simulink model "nmm2d"  (R2025a)
settings: Solver=ode15s  StartTime=0.0  StopTime=20  FixedStep=1e-3  MaxStep=ts_max  RelTol=1e-3  AbsTol=1e-4  EnableMultiTasking=on
values from neighbouring files (symbols this model uses):
  c = 0.05    [nmm2d_mInit.m]
  c_jointstop = 0.3 / (pi/180)    (= 17.1887338539)    [nmm2d_mInit.m]
  D12_F = 0.16    [nmm2d_mInit.m]
  D12_S = L_S    (= 0.5)    [nmm2d_mInit.m]
  D12_T = L_T    (= 0.5)    [nmm2d_mInit.m]
  D1G_F = 0.14    [nmm2d_mInit.m]
  D1G_HAT = 0.35    [nmm2d_mInit.m]
  D1G_S = 0.3    [nmm2d_mInit.m]
  D1G_T = 0.3    [nmm2d_mInit.m]
  DeltaThRef = 5e-3    (= 0.005)    [nmm2d_mInit.m]
  eref = 0.04    [nmm2d_mInit.m]
  FmaxVec = [FmaxSOL FmaxTA FmaxGAS FmaxVAS FmaxHAM FmaxGLU FmaxHFL               FmaxSOL FmaxTA FmaxGAS FmaxVAS FmaxHAM FmaxGLU FmaxHFL]'    [nmm2d_mInit.m]
  g = 9.81    [nmm2d_mInit.m]
  GainDeltaTheta = 2 /100*180/pi    (= 1.14591559026)    [nmm2d_cInit.m]
  GainGAS = 1.1/FmaxGAS    [nmm2d_cInit.m]
  GainGLU = 0.5/FmaxGLU    [nmm2d_cInit.m]
  GainHAM = 0.65/FmaxHAM    [nmm2d_cInit.m]
  GainHAMHFL = 4    [nmm2d_cInit.m]
  GainHFL = 0.5    [nmm2d_cInit.m]
  GainKneOverExt = 2    [nmm2d_cInit.m]
  GainSOL = 1.2/FmaxSOL    [nmm2d_cInit.m]
  GainSOLTA = 0.4/FmaxSOL    [nmm2d_cInit.m]
  GainTA = 1.1    [nmm2d_cInit.m]
  GainVAS = 1.2/FmaxVAS    [nmm2d_cInit.m]
  HAT_CG0 = [-D12_F; 0] + Rot120*[L_S;0] + Rot120*Rot230*[-L_T;0]            + Rot120*Rot230*Rot340*[D1G_HAT;0]    [nmm2d_cInit.m]
  In_F = 0.005    [nmm2d_mInit.m]
  In_HAT = 3    [nmm2d_mInit.m]
  In_S = 0.05    [nmm2d_mInit.m]
  In_T = 0.15    [nmm2d_mInit.m]
  K = 5    [nmm2d_mInit.m]
  k_gx = (2*(m_F+m_S+m_T)+m_HAT)*g/0.1    (= 7848)    [nmm2d_mInit.m]
  k_gy = (2*(m_F+m_S+m_T)+m_HAT)*g/0.01    (= 78480)    [nmm2d_mInit.m]
  k_pressure = m_HAT * 9.81 / DeltaThRef    (= 104967)    [nmm2d_mInit.m]
  K_swing = 0.25    [nmm2d_cInit.m]
  KneePh23Offset = 170*pi/180    (= 2.96705972839)    [nmm2d_cInit.m]
  L_F = 0.2    [nmm2d_mInit.m]
  L_HAT = 0.8    [nmm2d_mInit.m]
  L_S = 0.5    [nmm2d_mInit.m]
  L_T = 0.5    [nmm2d_mInit.m]
  LceOffsetHAM = 0.85    [nmm2d_cInit.m]
  LceOffsetHFL = 0.65    [nmm2d_cInit.m]
  LceOffsetTA = 1-0.5*w    [nmm2d_cInit.m]
  LongDelay = 0.020    (= 0.02)    [nmm2d_cInit.m]
  loptGAS = 0.05    [nmm2d_mInit.m]
  loptGLU = 0.11    [nmm2d_mInit.m]
  loptHAM = 0.10    (= 0.1)    [nmm2d_mInit.m]
  loptHFL = 0.11    [nmm2d_mInit.m]
  loptSOL = 0.04    [nmm2d_mInit.m]
  loptTA = 0.06    [nmm2d_mInit.m]
  loptVAS = 0.08    [nmm2d_mInit.m]
  loptVec = [loptSOL loptTA loptGAS loptVAS loptHAM loptGLU loptHFL               loptSOL loptTA loptGAS loptVAS loptHAM loptGLU loptHFL]'    [nmm2d_mInit.m]
  Lphi120 = 85*pi/180    (= 1.4835298642)    [nmm2d_cInit.m]
  Lphi230 = 175*pi/180    (= 3.05432619099)    [nmm2d_cInit.m]
  Lphi340 = 175*pi/180    (= 3.05432619099)    [nmm2d_cInit.m]
  lslackGAS = 0.40    (= 0.4)    [nmm2d_mInit.m]
  lslackGLU = 0.13    [nmm2d_mInit.m]
  lslackHAM = 0.31    [nmm2d_mInit.m]
  lslackHFL = 0.10    (= 0.1)    [nmm2d_mInit.m]
  lslackSOL = 0.26    [nmm2d_mInit.m]
  lslackTA = 0.24    [nmm2d_mInit.m]
  lslackVAS = 0.23    [nmm2d_mInit.m]
  lslackVec = [lslackSOL lslackTA lslackGAS lslackVAS lslackHAM lslackGLU lslackHFL                 lslackSOL lslackTA lslackGAS lslackVAS lslackHAM lslackGLU lslackHFL]'    [nmm2d_mInit.m]
  m_F = 1.25    [nmm2d_mInit.m]
  m_HAT = 53.5    [nmm2d_mInit.m]
  m_S = 3.5    [nmm2d_mInit.m]
  m_T = 8.5    [nmm2d_mInit.m]
  MidDelay = 0.010    (= 0.01)    [nmm2d_cInit.m]
  mu_slide = 0.8    [nmm2d_mInit.m]
  mu_stick = 0.9    [nmm2d_mInit.m]
  N = 1.5    [nmm2d_mInit.m]
  phi12_LowLimit = 70*pi/180    (= 1.2217304764)    [nmm2d_mInit.m]
  phi12_UpLimit = 130*pi/180    (= 2.26892802759)    [nmm2d_mInit.m]
  phi23_UpLimit = 175*pi/180    (= 3.05432619099)    [nmm2d_mInit.m]
  phi34_UpLimit = 230*pi/180    (= 4.01425727959)    [nmm2d_mInit.m]
  phimaxGASa = 110*pi/180    (= 1.91986217719)    [nmm2d_mInit.m]
  phimaxGASk = 140*pi/180    (= 2.44346095279)    [nmm2d_mInit.m]
  phimaxHAMk = 180*pi/180    (= 3.14159265359)    [nmm2d_mInit.m]
  phimaxSOL = 110*pi/180    (= 1.91986217719)    [nmm2d_mInit.m]
  phimaxTA = 80*pi/180    (= 1.3962634016)    [nmm2d_mInit.m]
  phimaxVAS = 165*pi/180    (= 2.87979326579)    [nmm2d_mInit.m]
  phirefGASa = 80*pi/180    (= 1.3962634016)    [nmm2d_mInit.m]
  phirefGASk = 165*pi/180    (= 2.87979326579)    [nmm2d_mInit.m]
  phirefGLU = 150*pi/180    (= 2.61799387799)    [nmm2d_mInit.m]
  phirefHAMh = 155*pi/180    (= 2.70526034059)    [nmm2d_mInit.m]
  phirefHAMk = 180*pi/180    (= 3.14159265359)    [nmm2d_mInit.m]
  phirefHFL = 180*pi/180    (= 3.14159265359)    [nmm2d_mInit.m]
  phirefSOL = 80*pi/180    (= 1.3962634016)    [nmm2d_mInit.m]
  phirefTA = 110*pi/180    (= 1.91986217719)    [nmm2d_mInit.m]
  phirefVAS = 125*pi/180    (= 2.18166156499)    [nmm2d_mInit.m]
  PosGainGG = 1/(30*pi/180)    (= 1.9098593171)    [nmm2d_cInit.m]
  preA = 0.01    [nmm2d_mInit.m]
  PreStimGAS = 0.01    [nmm2d_cInit.m]
  PreStimGG = 0.05    [nmm2d_cInit.m]
  PreStimGLU = 0.01    [nmm2d_cInit.m]
  PreStimHAM = 0.01    [nmm2d_cInit.m]
  PreStimHFL = 0.01    [nmm2d_cInit.m]
  PreStimSOL = 0.01    [nmm2d_cInit.m]
  PreStimTA = 0.01    [nmm2d_cInit.m]
  PreStimVAS = 0.08    [nmm2d_cInit.m]
  rGASa = 0.05    [nmm2d_mInit.m]
  rGASk = 0.05    [nmm2d_mInit.m]
  rGLU = 0.10    (= 0.1)    [nmm2d_mInit.m]
  rHAMh = 0.08    [nmm2d_mInit.m]
  rHAMk = 0.05    [nmm2d_mInit.m]
  rHFL = 0.10    (= 0.1)    [nmm2d_mInit.m]
  rhoGASa = 0.7    [nmm2d_mInit.m]
  rhoGASk = 0.7    [nmm2d_mInit.m]
  rhoGLU = 0.5    [nmm2d_mInit.m]
  rhoHAMh = 0.7    [nmm2d_mInit.m]
  rhoHAMk = 0.7    [nmm2d_mInit.m]
  rhoHFL = 0.5    [nmm2d_mInit.m]
  rhoSOL = 0.5    [nmm2d_mInit.m]
  rhoTA = 0.7    [nmm2d_mInit.m]
  rhoVAS = 0.7    [nmm2d_mInit.m]
  Rphi120 = 90*pi/180    (= 1.57079632679)    [nmm2d_cInit.m]
  Rphi230 = 175*pi/180    (= 3.05432619099)    [nmm2d_cInit.m]
  Rphi340 = 140*pi/180    (= 2.44346095279)    [nmm2d_cInit.m]
  rSOL = 0.05    [nmm2d_mInit.m]
  rTA = 0.04    [nmm2d_mInit.m]
  rVAS = 0.06    [nmm2d_mInit.m]
  ... (+12 more)
undefined symbols (not defined in the file or in its folder): sgn, X, Y, Z
libraries: sm_lib x70, nesl_utility x67, simulink x27, simulink_extras x6
(part 4 of 5)

== system nmm2d/Body Mechanics Layer/body sensor2 ==
  Frame Sensor : sm_lib/Frames and Transforms/Transform Sensor  MeasurementFrame=World  RotationSequence=XYX  SenseAngle=off  SenseAxis=off  SenseQ=off  SenseR=off  SenseRotationSequence=off  SenseOmegaX=off  SenseOmegaY=off  SenseOmegaZ=off  SenseOmega=off  SenseQDot=off  SenseRDot=off  SenseRotationSequenceDot=off  SenseAlphaX=off  SenseAlphaY=off  SenseAlphaZ=off  SenseAlpha=off  SenseQDDot=off  SenseRDDot=off  SenseX=on  SenseY=on  SenseZ=on  SenseXYZ=off  SenseRad=off  SenseAzim=off  SenseDist=off  SenseInc=off  SenseXDot=on  SenseYDot=on  SenseZDot=on  SenseXYZDot=off  SenseRadDot=off  SenseAzimDot=off  SenseDistDot=off  SenseIncDot=off  SenseXDDot=off  SenseYDDot=off  SenseZDDot=off  SenseXYZDDot=off  SenseRadDDot=off  SenseAzimDDot=off  SenseDistDDot=off  SenseIncDDot=off
  Mux : Mux  Inputs=3
  Mux1 : Mux  Inputs=3
  PS-Simulink Converter : nesl_utility/PS-Simulink Converter  PhysicalDomain=network_engine_domain  SubClassName=ps_output  LeftPortType=input  RightPortType=output  PseudoPeriodic=off  Frequencies=[]  VectorFormat=1-D array  Unit=m  AffineConversion=off
  PS-Simulink Converter1 : nesl_utility/PS-Simulink Converter  PhysicalDomain=network_engine_domain  SubClassName=ps_output  LeftPortType=input  RightPortType=output  PseudoPeriodic=off  Frequencies=[]  VectorFormat=1-D array  Unit=m  AffineConversion=off
  PS-Simulink Converter2 : nesl_utility/PS-Simulink Converter  PhysicalDomain=network_engine_domain  SubClassName=ps_output  LeftPortType=input  RightPortType=output  PseudoPeriodic=off  Frequencies=[]  VectorFormat=1-D array  Unit=m/s  AffineConversion=off
  PS-Simulink Converter3 : nesl_utility/PS-Simulink Converter  PhysicalDomain=network_engine_domain  SubClassName=ps_output  LeftPortType=input  RightPortType=output  PseudoPeriodic=off  Frequencies=[]  VectorFormat=1-D array  Unit=m/s  AffineConversion=off
  PS-Simulink Converter4 : nesl_utility/PS-Simulink Converter  PhysicalDomain=network_engine_domain  SubClassName=ps_output  LeftPortType=input  RightPortType=output  PseudoPeriodic=off  Frequencies=[]  VectorFormat=1-D array  Unit=m  AffineConversion=off
  PS-Simulink Converter5 : nesl_utility/PS-Simulink Converter  PhysicalDomain=network_engine_domain  SubClassName=ps_output  LeftPortType=input  RightPortType=output  PseudoPeriodic=off  Frequencies=[]  VectorFormat=1-D array  Unit=m/s  AffineConversion=off
  World Frame : sm_lib/Frames and Transforms/World Frame
  frame : PMIOPort  Side=Left
  p [m x3] : Outport
  v [m/s x3] : Outport  Port=2
  wires:
  PS-Simulink Converter1/1 -> Mux/2
  PS-Simulink Converter/1 -> Mux/1
  PS-Simulink Converter2/1 -> Mux1/1
  PS-Simulink Converter3/1 -> Mux1/2
  Mux1/1 -> v [m/s x3]/1
  Mux/1 -> p [m x3]/1
  PS-Simulink Converter4/1 -> Mux/3
  PS-Simulink Converter5/1 -> Mux1/3
  connections:
  Frame Sensor/RConn1 -- frame/RConn1
  World Frame/RConn1 -- Frame Sensor/LConn1
  Frame Sensor/RConn2 -- PS-Simulink Converter/LConn1
  PS-Simulink Converter1/LConn1 -- Frame Sensor/RConn3
  PS-Simulink Converter2/LConn1 -- Frame Sensor/RConn5
  PS-Simulink Converter3/LConn1 -- Frame Sensor/RConn6
  PS-Simulink Converter4/LConn1 -- Frame Sensor/RConn4
  PS-Simulink Converter5/LConn1 -- Frame Sensor/RConn7

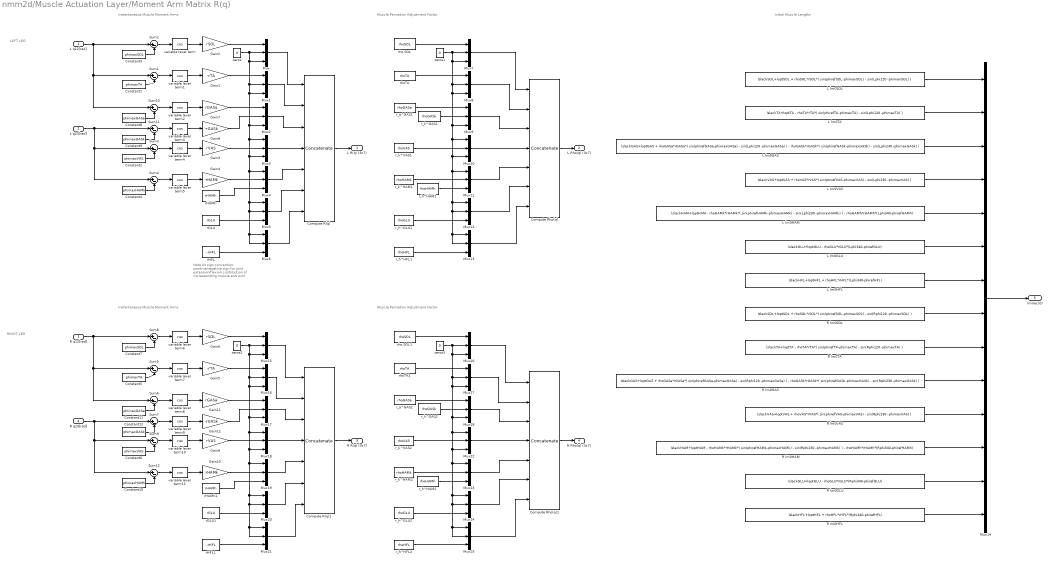
== system nmm2d/Muscle Actuation Layer/Moment Arm Matrix R(q) ==
  note: LEFT LEG
  note: Muscle Pennation Adjustment Factor
  note: Initial Muscle Lengths
  note: Instantaneous Muscle Moment Arms
  note: Note on sign convention:
      | positive/negative sign for
      | joint extension/flexion contribution
      | of corresponding muscle and joint
  note: Instantaneous Muscle Moment Arms
  note: RIGHT LEG
  note: Muscle Pennation Adjustment Factor
  L q12[rad] : Inport
  L q23[rad] : Inport  Port=2
  R q12[rad] : Inport  Port=3
  R q23[rad] : Inport  Port=4
  Compute R(q) : Concatenate  NumInputs=7  Mode=Multidimensional array  ConcatenateDimension=2
  Compute R(q)1 : Concatenate  NumInputs=7  Mode=Multidimensional array  ConcatenateDimension=2
  Compute Rho(q) : Concatenate  NumInputs=7  Mode=Multidimensional array  ConcatenateDimension=2
  Compute Rho(q)1 : Concatenate  NumInputs=7  Mode=Multidimensional array  ConcatenateDimension=2
  Constant1 : Constant  Value=phimaxTA
  Constant10 : Constant  Value=phimaxHAMk
  Constant11 : Constant  Value=phimaxGASa
  Constant12 : Constant  Value=phimaxGASk
  Constant2 : Constant  Value=phimaxVAS
  Constant3 : Constant  Value=phimaxSOL
  Constant4 : Constant  Value=phimaxHAMk
  Constant5 : Constant  Value=phimaxTA
  Constant6 : Constant  Value=phimaxVAS
  Constant7 : Constant  Value=phimaxSOL
  Constant8 : Constant  Value=phimaxGASa
  Constant9 : Constant  Value=phimaxGASk
  Gain1 : Gain  Gain=-rTA
  Gain10 : Gain  Gain=-rHAMk
  Gain11 : Gain  Gain=rGASa
  Gain12 : Gain  Gain=-rGASk
  Gain2 : Gain  Gain=rSOL
  Gain3 : Gain  Gain=rVAS
  Gain4 : Gain  Gain=-rHAMk
  Gain5 : Gain  Gain=-rTA
  Gain6 : Gain  Gain=rSOL
  Gain7 : Gain  Gain=rGASa
  Gain8 : Gain  Gain=-rGASk
  Gain9 : Gain  Gain=rVAS
  L lm0GAS : Constant  Value=lslackGAS+loptGAS + rhoGASa*rGASa*( sin(phirefGASa-phimaxGASa) - sin(Lphi120 -phimaxGASa) ) - rhoGASk*rGASk*( sin(phirefGASk-phimaxGASk) - sin(Lphi230 -phimaxGASk) )
  L lm0GLU : Constant  Value=lslackGLU+loptGLU - rhoGLU*rGLU*(Lphi340-phirefGLU)
  L lm0HAM : Constant  Value=lslackHAM+loptHAM - rhoHAMk*rHAMk*( sin(phirefHAMk-phimaxHAMk) - sin(Lphi230 -phimaxHAMk) ) - rhoHAMh*rHAMh*(Lphi340-phirefHAMh)
  L lm0HFL : Constant  Value=lslackHFL+loptHFL + rhoHFL*rHFL*(Lphi340-phirefHFL)
  L lm0SOL : Constant  Value=lslackSOL+loptSOL + rhoSOL*rSOL*( sin(phirefSOL-phimaxSOL) - sin(Lphi120 -phimaxSOL) )
  L lm0TA : Constant  Value=lslackTA+loptTA - rhoTA*rTA*( sin(phirefTA-phimaxTA) - sin(Lphi120 -phimaxTA) )
  L lm0VAS : Constant  Value=lslackVAS+loptVAS + rhoVAS*rVAS*( sin(phirefVAS-phimaxVAS) - sin(Lphi230 -phimaxVAS) )
  Mux{,1..13,15..28} (28 alike) : Mux  Inputs=3
  Mux14 : Mux  Inputs=14
  R lm0GAS : Constant  Value=lslackGAS+loptGAS + rhoGASa*rGASa*( sin(phirefGASa-phimaxGASa) - sin(Rphi120 -phimaxGASa) ) - rhoGASk*rGASk*( sin(phirefGASk-phimaxGASk) - sin(Rphi230 -phimaxGASk) )
  R lm0GLU : Constant  Value=lslackGLU+loptGLU - rhoGLU*rGLU*(Rphi340-phirefGLU)
  R lm0HAM : Constant  Value=lslackHAM+loptHAM - rhoHAMk*rHAMk*( sin(phirefHAMk-phimaxHAMk) - sin(Rphi230 -phimaxHAMk) ) - rhoHAMh*rHAMh*(Rphi340-phirefHAMh)
  R lm0HFL : Constant  Value=lslackHFL+loptHFL + rhoHFL*rHFL*(Rphi340-phirefHFL)
  R lm0SOL : Constant  Value=lslackSOL+loptSOL + rhoSOL*rSOL*( sin(phirefSOL-phimaxSOL) - sin(Rphi120 -phimaxSOL) )
  R lm0TA : Constant  Value=lslackTA+loptTA - rhoTA*rTA*( sin(phirefTA-phimaxTA) - sin(Rphi120 -phimaxTA) )
  R lm0VAS : Constant  Value=lslackVAS+loptVAS + rhoVAS*rVAS*( sin(phirefVAS-phimaxVAS) - sin(Rphi230 -phimaxVAS) )
  Sum{1..12} (12 alike) : Sum  Inputs=|+-
  rGLU : Constant  Value=rGLU
  rGLU1 : Constant  Value=rGLU
  rHAMh : Constant  Value=rHAMh
  rHAMh1 : Constant  Value=rHAMh
  rHFL : Constant  Value=-rHFL
  rHFL1 : Constant  Value=-rHFL
  r_a^GAS1 : Constant  Value=rhoGASa
  r_a^GAS2 : Constant  Value=rhoGASa
  r_h^GLU1 : Constant  Value=rhoGLU
  r_h^GLU2 : Constant  Value=rhoGLU
  r_h^HAM1 : Constant  Value=rhoHAMh
  r_h^HAM2 : Constant  Value=rhoHAMh
  r_h^HFL1 : Constant  Value=rhoHFL
  r_h^HFL2 : Constant  Value=rhoHFL
  r_k^GAS1 : Constant  Value=rhoGASk
  r_k^GAS2 : Constant  Value=rhoGASk
  r_k^HAM1 : Constant  Value=rhoHAMk
  r_k^HAM2 : Constant  Value=rhoHAMk
  r_k^VAS1 : Constant  Value=rhoVAS
  r_k^VAS2 : Constant  Value=rhoVAS
  rho SOL : Constant  Value=rhoSOL
  rho SOL1 : Constant  Value=rhoSOL
  rhoTA : Constant  Value=rhoTA
  rhoTA1 : Constant  Value=rhoTA
  variable lever term{,1..11} (12 alike) : Trigonometry  Operator=cos
  zeros{,1..3} (4 alike) : Constant  Value=0
  L R(q) (3x7) : Outport
  L Rho(q) (3x7) : Outport  Port=2
  R R(q) (3x7) : Outport  Port=3
  R Rho(q) (3x7) : Outport  Port=4
  lmVec(0) : Outport  Port=5
  wires:
  Compute Rho(q)/1 -> L Rho(q) (3x7)/1
  rho SOL/1 -> Mux7/1
  Mux7/1 -> Compute Rho(q)/1
  r_k^GAS1/1 -> Mux9/2
  r_k^HAM1/1 -> Mux11/2
  r_k^VAS1/1 -> Mux10/2
  Mux13/1 -> Compute Rho(q)/7
  Mux8/1 -> Compute Rho(q)/2
  r_h^HAM1/1 -> Mux11/3
  Mux12/1 -> Compute Rho(q)/6
  r_h^GLU1/1 -> Mux12/3
  r_h^HFL1/1 -> Mux13/3
  Mux10/1 -> Compute Rho(q)/4
  rhoTA/1 -> Mux8/1
  Mux9/1 -> Compute Rho(q)/3
  zeros1/1 -> Mux7/2, Mux7/3, Mux8/2, Mux8/3, Mux9/3, Mux10/1, Mux10/3, Mux11/1, Mux12/1, Mux12/2, Mux13/2, Mux13/1
  r_a^GAS1/1 -> Mux9/1
  Mux11/1 -> Compute Rho(q)/5
  L lm0VAS/1 -> Mux14/4
  L lm0SOL/1 -> Mux14/1
  L lm0GAS/1 -> Mux14/3
  L q23[rad]/1 -> Sum11/1, Sum3/1, Sum4/1
  Sum4/1 -> variable lever term5/1
  Constant4/1 -> Sum4/2
  variable lever term5/1 -> Gain4/1
  Constant3/1 -> Sum2/2
  variable lever term/1 -> Gain2/1
  Constant2/1 -> Sum3/2
  variable lever term4/1 -> Gain3/1
  Mux/1 -> Compute R(q)/1
  Gain4/1 -> Mux4/2
  Mux6/1 -> Compute R(q)/7
  L lm0HAM/1 -> Mux14/5
  Gain2/1 -> Mux/1
  Sum3/1 -> variable lever term4/1
  Compute R(q)/1 -> L R(q) (3x7)/1
  Mux2/1 -> Compute R(q)/3
  Gain7/1 -> Mux2/1
  Mux5/1 -> Compute R(q)/6
  Gain8/1 -> Mux2/2
  Mux1/1 -> Compute R(q)/2
  rGLU/1 -> Mux5/3
  zeros/1 -> Mux/2, Mux/3, Mux1/2, Mux1/3, Mux2/3, Mux3/1, Mux3/3, Mux4/1, Mux5/1, Mux5/2, Mux6/2, Mux6/1
  Gain3/1 -> Mux3/2
  Mux4/1 -> Compute R(q)/5
  Sum2/1 -> variable lever term/1
  rHAMh/1 -> Mux4/3
  rHFL/1 -> Mux6/3
  Mux3/1 -> Compute R(q)/4
  Sum1/1 -> variable lever term1/1
  variable lever term1/1 -> Gain1/1
  Gain1/1 -> Mux1/1
  L lm0GLU/1 -> Mux14/6
  L lm0HFL/1 -> Mux14/7
  Mux14/1 -> lmVec(0)/1
  variable lever term3/1 -> Gain8/1
  L lm0TA/1 -> Mux14/2
  Constant9/1 -> Sum11/2
  L q12[rad]/1 -> Sum2/1, Sum1/1, Sum10/1
  variable lever term2/1 -> Gain7/1
  Constant8/1 -> Sum10/2
  Constant1/1 -> Sum1/2
  Sum10/1 -> variable lever term2/1
  Sum11/1 -> variable lever term3/1
  Gain10/1 -> Mux19/2
  Constant7/1 -> Sum8/2
  Sum6/1 -> variable lever term8/1
  rHAMh1/1 -> Mux19/3
  Sum9/1 -> variable lever term10/1
  Sum8/1 -> variable lever term6/1
  rHFL1/1 -> Mux21/3
  Constant5/1 -> Sum5/2
  variable lever term8/1 -> Gain11/1
  Gain5/1 -> Mux16/1
  zeros2/1 -> Mux21/1, Mux21/2, Mux20/2, Mux20/1, Mux19/1, Mux18/3, Mux18/1, Mux17/3, Mux16/3, Mux16/2, Mux15/3, Mux15/2
  variable lever term7/1 -> Gain5/1
  Gain12/1 -> Mux17/2
  variable lever term11/1 -> Gain10/1
  Constant11/1 -> Sum6/2
  Sum12/1 -> variable lever term11/1
  Constant6/1 -> Sum9/2
  variable lever term10/1 -> Gain9/1
  Gain11/1 -> Mux17/1
  variable lever term6/1 -> Gain6/1
  R q12[rad]/1 -> Sum6/1, Sum5/1, Sum8/1
  R q23[rad]/1 -> Sum12/1, Sum9/1, Sum7/1
  variable lever term9/1 -> Gain12/1
  Gain9/1 -> Mux18/2
  Sum7/1 -> variable lever term9/1
  Constant10/1 -> Sum12/2
  Gain6/1 -> Mux15/1
  Sum5/1 -> variable lever term7/1
  Constant12/1 -> Sum7/2
  rGLU1/1 -> Mux20/3
  r_a^GAS2/1 -> Mux28/1
  zeros3/1 -> Mux25/1, Mux25/2, Mux24/2, Mux24/1, Mux23/1, Mux22/3, Mux22/1, Mux28/3, Mux27/3, Mux27/2, Mux26/3, Mux26/2
  rhoTA1/1 -> Mux27/1
  r_h^HFL2/1 -> Mux25/3
  r_h^GLU2/1 -> Mux24/3
  r_h^HAM2/1 -> Mux23/3
  r_k^VAS2/1 -> Mux22/2
  r_k^HAM2/1 -> Mux23/2
  r_k^GAS2/1 -> Mux28/2
  rho SOL1/1 -> Mux26/1
  R lm0SOL/1 -> Mux14/8
  R lm0TA/1 -> Mux14/9
  R lm0VAS/1 -> Mux14/11
  R lm0GAS/1 -> Mux14/10
  R lm0HAM/1 -> Mux14/12
  R lm0GLU/1 -> Mux14/13
  R lm0HFL/1 -> Mux14/14
  Compute Rho(q)1/1 -> R Rho(q) (3x7)/1
  Mux22/1 -> Compute Rho(q)1/4
  Mux26/1 -> Compute Rho(q)1/1
  Mux27/1 -> Compute Rho(q)1/2
  Mux28/1 -> Compute Rho(q)1/3
  Mux23/1 -> Compute Rho(q)1/5
  Mux24/1 -> Compute Rho(q)1/6
  Mux25/1 -> Compute Rho(q)1/7
  Compute R(q)1/1 -> R R(q) (3x7)/1
  Mux18/1 -> Compute R(q)1/4
  Mux15/1 -> Compute R(q)1/1
  Mux16/1 -> Compute R(q)1/2
  Mux17/1 -> Compute R(q)1/3
  Mux19/1 -> Compute R(q)1/5
  Mux20/1 -> Compute R(q)1/6
  Mux21/1 -> Compute R(q)1/7

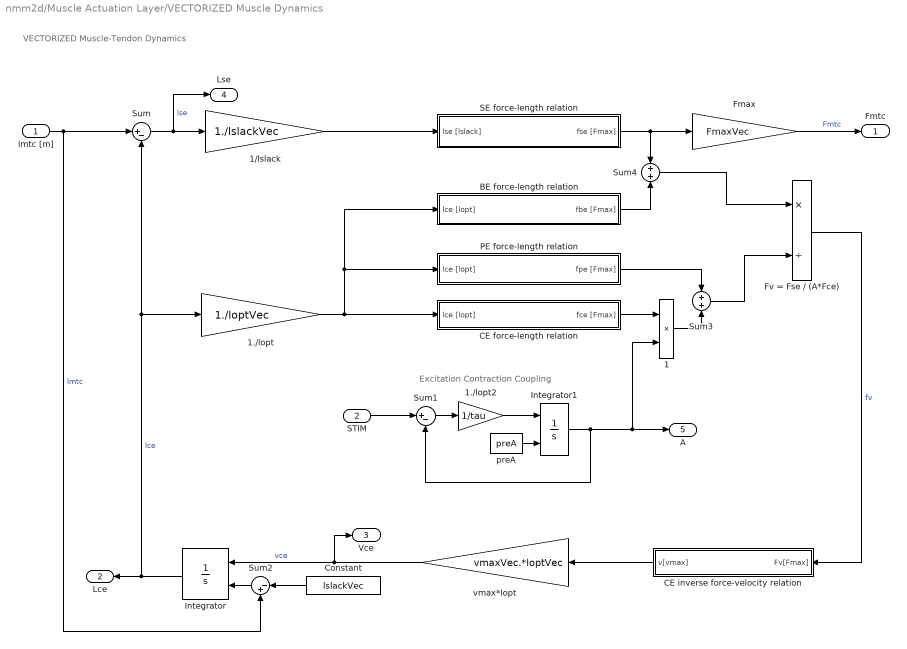
== system nmm2d/Muscle Actuation Layer/VECTORIZED Muscle Dynamics ==
  note: Excitation Contraction Coupling
  note: VECTORIZED Muscle-Tendon Dynamics
  lmtc [m] : Inport
  STIM : Inport  Port=2
  1 : Product  Inputs=**  InputSameDT=on  SaturateOnIntegerOverflow=on  OutDataTypeStr=Inherit: Same as first input
  1./lopt : Gain  Gain=1./loptVec  SaturateOnIntegerOverflow=on  OutDataTypeStr=Inherit: Same as input  ParamDataTypeStr=Inherit: Same as input
  1./lopt2 : Gain  Gain=1/tau  SaturateOnIntegerOverflow=on  OutDataTypeStr=Inherit: Same as input  ParamDataTypeStr=Inherit: Same as input
  1/lslack : Gain  Gain=1./lslackVec  SaturateOnIntegerOverflow=on  OutDataTypeStr=Inherit: Same as input  ParamDataTypeStr=Inherit: Same as input
  BE force-length relation : Subsystem
  CE force-length relation : Subsystem
  CE inverse force-velocity relation : Subsystem
  Constant : Constant  Value=lslackVec
  Fmax : Gain  Gain=FmaxVec  SaturateOnIntegerOverflow=on  OutDataTypeStr=Inherit: Same as input  ParamDataTypeStr=Inherit: Same as input
  Fv = Fse / (A*Fce) : Product  Inputs=*/  InputSameDT=on  SaturateOnIntegerOverflow=on  OutDataTypeStr=Inherit: Same as first input
  Integrator : Integrator  InitialConditionSource=external  LowerSaturationLimit=0.05
  Integrator1 : Integrator  InitialConditionSource=external  LowerSaturationLimit=0.05
  PE force-length relation : Subsystem
  SE force-length relation : Subsystem
  Sum : Sum  Inputs=|+-  InputSameDT=on  SaturateOnIntegerOverflow=on  OutDataTypeStr=Inherit: Same as first input
  Sum1 : Sum  Inputs=|+-  InputSameDT=on  SaturateOnIntegerOverflow=on  OutDataTypeStr=Inherit: Same as first input
  Sum2 : Sum  Inputs=|-+  InputSameDT=on  SaturateOnIntegerOverflow=on  OutDataTypeStr=Inherit: Same as first input
  Sum3 : Sum  InputSameDT=on  SaturateOnIntegerOverflow=on  OutDataTypeStr=Inherit: Same as first input
  Sum4 : Sum  InputSameDT=on  SaturateOnIntegerOverflow=on  OutDataTypeStr=Inherit: Same as first input
  preA : Constant  Value=preA
  vmax*lopt : Gain  Gain=vmaxVec.*loptVec  SaturateOnIntegerOverflow=on  OutDataTypeStr=Inherit: Same as input  ParamDataTypeStr=Inherit: Same as input
  Fmtc : Outport  InitialOutput=0
  Lce : Outport  Port=2  InitialOutput=0
  Vce : Outport  Port=3  InitialOutput=0
  Lse : Outport  Port=4  InitialOutput=0
  A : Outport  Port=5  InitialOutput=0
  wires:
  1./lopt2/1 -> Integrator1/1
  Sum1/1 -> 1./lopt2/1
  CE inverse force-velocity relation/1(v[vmax]) -> vmax*lopt/1
  Fv = Fse / (A*Fce)/1 -> CE inverse force-velocity relation/1(Fv[Fmax])  "fv"
  Sum3/1 -> Fv = Fse / (A*Fce)/2
  Sum4/1 -> Fv = Fse / (A*Fce)/1
  SE force-length relation/1(fse [Fmax]) -> Fmax/1, Sum4/1
  preA/1 -> Integrator1/2
  STIM/1 -> Sum1/1
  Integrator1/1 -> Sum1/2, 1/2, A/1
  BE force-length relation/1(fbe [Fmax]) -> Sum4/2
  1/1 -> Sum3/2
  PE force-length relation/1(fpe [Fmax]) -> Sum3/1
  CE force-length relation/1(fce [Fmax]) -> 1/1
  Constant/1 -> Sum2/1
  Sum2/1 -> Integrator/2
  1/lslack/1 -> SE force-length relation/1(lse [lslack])
  Fmax/1 -> Fmtc/1  "Fmtc"
  lmtc [m]/1 -> Sum/1, Sum2/2  "lmtc"
  vmax*lopt/1 -> Vce/1, Integrator/1  "vce"
  1./lopt/1 -> CE force-length relation/1(lce [lopt]), BE force-length relation/1(lce [lopt]), PE force-length relation/1(lce [lopt])
  Sum/1 -> Lse/1, 1/lslack/1  "lse"
  Integrator/1 -> Lce/1, 1./lopt/1, Sum/2  "lce"

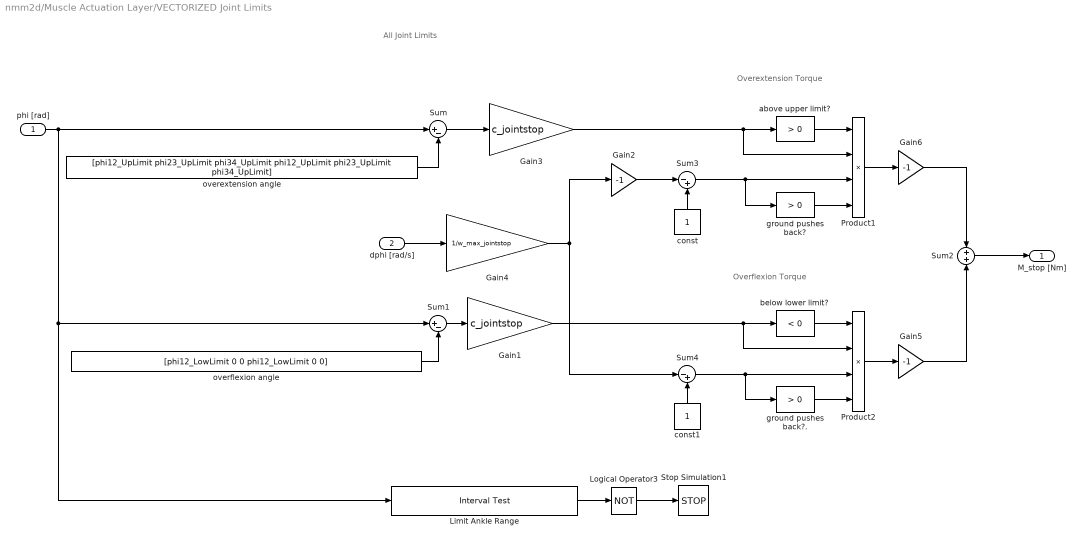
== system nmm2d/Muscle Actuation Layer/VECTORIZED Joint Limits ==
  note: Overextension Torque
  note: All Joint Limits
  note: Overflexion Torque
  phi [rad] : Inport
  dphi [rad/s] : Inport  Port=2
  Gain1 : Gain  Gain=c_jointstop
  Gain2 : Gain  Gain=-1
  Gain3 : Gain  Gain=c_jointstop
  Gain4 : Gain  Gain=1/w_max_jointstop
  Gain5 : Gain  Gain=-1
  Gain6 : Gain  Gain=-1
  Limit Ankle Range : simulink/Logic and Bit Operations/Interval Test  IntervalClosedRight=on  uplimit=[phi12_UpLimit + 40*pi/180, 185*pi/180, phi34_UpLimit + 30*pi/180 phi12_UpLimit + 40*pi/180, 185*pi/180, phi34_UpLimit + 30*pi/180]  IntervalClosedLeft=on  lowlimit=[phi12_LowLimit - 40*pi/180, 40*pi/180, 10*pi/180 phi12_LowLimit - 40*pi/180, 40*pi/180, 10*pi/180]  OutDataTypeStr=boolean
      settings: AttributesFormatString=|
      | Lower limits: %<lowlimit>
      | Upper limits: %<uplimit>
  Logical Operator3 : Logic  Operator=NOT  AllPortsSameDT=off  OutDataTypeStr=boolean
  Product1 : Product  Inputs=4
  Product2 : Product  Inputs=4
  Stop Simulation1 : Stop
  Sum : Sum  Inputs=|+-
  Sum1 : Sum  Inputs=|+-
  Sum2 : Sum
  Sum3 : Sum  Inputs=|-+
  Sum4 : Sum  Inputs=|-+
  above upper limit? : simulink/Logic and Bit Operations/Compare To Zero  relop=>  OutDataTypeStr=boolean  ZeroCross=off
  below lower limit? : simulink/Logic and Bit Operations/Compare To Zero  relop=<  OutDataTypeStr=boolean  ZeroCross=off
  const : Constant
  const1 : Constant
  ground pushes back? : simulink/Logic and Bit Operations/Compare To Zero  relop=>  OutDataTypeStr=boolean  ZeroCross=off
  ground pushes back?. : simulink/Logic and Bit Operations/Compare To Zero  relop=>  OutDataTypeStr=boolean  ZeroCross=off
  overextension angle : Constant  Value=[phi12_UpLimit phi23_UpLimit phi34_UpLimit phi12_UpLimit phi23_UpLimit phi34_UpLimit]
  overflexion angle : Constant  Value=[phi12_LowLimit 0 0 phi12_LowLimit 0 0]
  M_stop [Nm] : Outport
  wires:
  Logical Operator3/1 -> Stop Simulation1/1
  Limit Ankle Range/1 -> Logical Operator3/1
  Gain6/1 -> Sum2/1
  Gain2/1 -> Sum3/1
  Sum2/1 -> M_stop [Nm]/1
  overflexion angle/1 -> Sum1/2
  Sum1/1 -> Gain1/1
  Sum/1 -> Gain3/1
  phi [rad]/1 -> Sum/1, Sum1/1, Limit Ankle Range/1
  overextension angle/1 -> Sum/2
  dphi [rad/s]/1 -> Gain4/1
  const/1 -> Sum3/2
  Sum3/1 -> Product1/3, ground pushes back?/1
  Gain3/1 -> Product1/2, above upper limit?/1
  ground pushes back?/1 -> Product1/4
  above upper limit?/1 -> Product1/1
  Product1/1 -> Gain6/1
  Product2/1 -> Gain5/1
  below lower limit?/1 -> Product2/1
  ground pushes back?./1 -> Product2/4
  Gain1/1 -> below lower limit?/1, Product2/2
  Sum4/1 -> ground pushes back?./1, Product2/3
  const1/1 -> Sum4/2
  Gain4/1 -> Sum4/1, Gain2/1
  Gain5/1 -> Sum2/2

== system nmm2d/Neural Control Layer/Cross Influence Detection ==
  note: right leg is leading
  note: left leg is leading
  note: Double Support Cross Influences
  LStance : Inport
  RStance : Inport  Port=2
  DSup ends : HitCross  HitCrossingOffset=0.5  HitCrossingDirection=falling  ZeroCross=off
  Double Support? : Logic  AllPortsSameDT=off
  Double Support?1 : Logic  AllPortsSameDT=off
  Double Support?4 : Logic  AllPortsSameDT=off
  Flight? : Logic  Operator=NOR  AllPortsSameDT=off
  LLeg starts DSup : HitCross  HitCrossingOffset=0.5  HitCrossingDirection=rising  ZeroCross=off
  Memory : Memory
  Memory3 : Memory
  RLeg starts DSup : HitCross  HitCrossingOffset=0.5  HitCrossingDirection=rising  ZeroCross=off
  S-R Flip-Flop : simulink_extras/Flip Flops/S-R Flip-Flop  initial_condition=0
  S-R Flip-Flop1 : simulink_extras/Flip Flops/S-R Flip-Flop  initial_condition=0
  Terminator1 : Terminator
  Terminator2 : Terminator
  RonL : Outport
  Flight : Outport  Port=2
  LonR : Outport  Port=3
  wires:
  S-R Flip-Flop/2 -> Terminator1/1
  Double Support?/1 -> DSup ends/1, Double Support?1/1, Double Support?4/2
  S-R Flip-Flop/1 -> LonR/1
  S-R Flip-Flop1/2 -> Terminator2/1
  LStance/1 -> Memory3/1, Double Support?/1, Flight?/1
  RStance/1 -> Memory/1, Double Support?/2, Flight?/2
  S-R Flip-Flop1/1 -> RonL/1
  Memory/1 -> RLeg starts DSup/1
  RLeg starts DSup/1 -> Double Support?1/2
  Double Support?1/1 -> S-R Flip-Flop1/1
  Memory3/1 -> LLeg starts DSup/1
  LLeg starts DSup/1 -> Double Support?4/1
  Double Support?4/1 -> S-R Flip-Flop/1
  DSup ends/1 -> S-R Flip-Flop/2, S-R Flip-Flop1/2
  Flight?/1 -> Flight/1

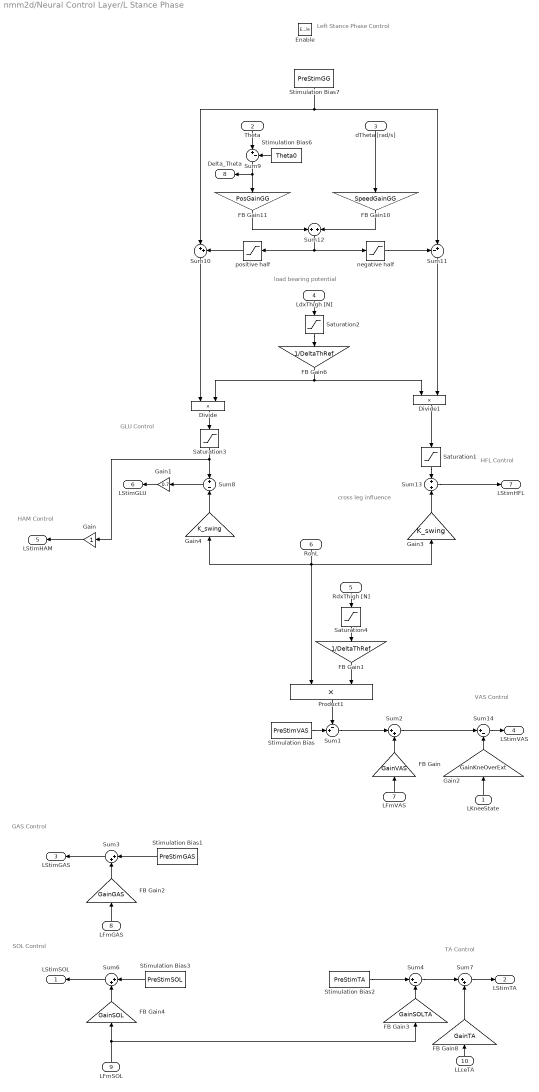
== system nmm2d/Neural Control Layer/L Stance Phase ==
  note: GLU Control
  note: SOL Control
  note: TA Control
  note: GAS Control
  note: VAS Control
  note: Left Stance Phase Control
  note: HAM Control
  note: cross leg influence
  note: HFL Control
  note: load bearing potential
  LKneeState : Inport
  Theta : Inport  Port=2
  dTheta [rad/s] : Inport  Port=3
  LdxThigh [N] : Inport  Port=4
  RdxThigh [N] : Inport  Port=5
  RonL : Inport  Port=6
  LFmVAS : Inport  Port=7
  LFmGAS : Inport  Port=8
  LFmSOL : Inport  Port=9
  LLceTA : Inport  Port=10
  Enable : EnablePort  StatesWhenEnabling=reset
  Divide : Product
  Divide1 : Product
  FB Gain : Gain  Gain=GainVAS  SaturateOnIntegerOverflow=on  OutDataTypeStr=Inherit: Same as input  ParamDataTypeStr=Inherit: Same as input
  FB Gain1 : Gain  Gain=1/DeltaThRef  SaturateOnIntegerOverflow=on  OutDataTypeStr=Inherit: Same as input  ParamDataTypeStr=Inherit: Same as input
  FB Gain10 : Gain  Gain=SpeedGainGG  SaturateOnIntegerOverflow=on  OutDataTypeStr=Inherit: Same as input  ParamDataTypeStr=Inherit: Same as input
  FB Gain11 : Gain  Gain=PosGainGG  SaturateOnIntegerOverflow=on  OutDataTypeStr=Inherit: Same as input  ParamDataTypeStr=Inherit: Same as input
  FB Gain2 : Gain  Gain=GainGAS  SaturateOnIntegerOverflow=on  OutDataTypeStr=Inherit: Same as input  ParamDataTypeStr=Inherit: Same as input
  FB Gain3 : Gain  Gain=GainSOLTA  SaturateOnIntegerOverflow=on  OutDataTypeStr=Inherit: Same as input  ParamDataTypeStr=Inherit: Same as input
  FB Gain4 : Gain  Gain=GainSOL  SaturateOnIntegerOverflow=on  OutDataTypeStr=Inherit: Same as input  ParamDataTypeStr=Inherit: Same as input
  FB Gain6 : Gain  Gain=1/DeltaThRef  SaturateOnIntegerOverflow=on  OutDataTypeStr=Inherit: Same as input  ParamDataTypeStr=Inherit: Same as input
  FB Gain8 : Gain  Gain=GainTA  SaturateOnIntegerOverflow=on  OutDataTypeStr=Inherit: Same as input  ParamDataTypeStr=Inherit: Same as input
  Gain : Gain
  Gain1 : Gain  Gain=0.7
  Gain2 : Gain  Gain=GainKneOverExt
  Gain3 : Gain  Gain=K_swing
  Gain4 : Gain  Gain=K_swing
  Product1 : Product  RndMeth=Zero
  Saturation1 : Saturate  UpperLimit=1  LowerLimit=0  ZeroCross=off
  Saturation2 : Saturate  UpperLimit=inf  LowerLimit=0  ZeroCross=off
  Saturation3 : Saturate  UpperLimit=1  LowerLimit=0  ZeroCross=off
  Saturation4 : Saturate  UpperLimit=inf  LowerLimit=0  ZeroCross=off
  Stimulation Bias : Constant  Value=PreStimVAS
  Stimulation Bias1 : Constant  Value=PreStimGAS
  Stimulation Bias2 : Constant  Value=PreStimTA
  Stimulation Bias3 : Constant  Value=PreStimSOL
  Stimulation Bias6 : Constant  Value=Theta0
  Stimulation Bias7 : Constant  Value=PreStimGG
  Sum1 : Sum  Inputs=-+|  InputSameDT=on  SaturateOnIntegerOverflow=on  OutDataTypeStr=Inherit: Same as first input
  Sum{2..3,6..7,10} (5 alike) : Sum  Inputs=|++  InputSameDT=on  SaturateOnIntegerOverflow=on  OutDataTypeStr=Inherit: Same as first input
  Sum11 : Sum  Inputs=-+|  InputSameDT=on  SaturateOnIntegerOverflow=on  OutDataTypeStr=Inherit: Same as first input
  Sum12 : Sum  InputSameDT=on  SaturateOnIntegerOverflow=on  OutDataTypeStr=Inherit: Same as first input
  Sum13 : Sum  InputSameDT=on  SaturateOnIntegerOverflow=on  OutDataTypeStr=Inherit: Same as first input
  Sum14 : Sum  Inputs=|+-  InputSameDT=on  SaturateOnIntegerOverflow=on  OutDataTypeStr=Inherit: Same as first input
  Sum4 : Sum  Inputs=|+-  InputSameDT=on  SaturateOnIntegerOverflow=on  OutDataTypeStr=Inherit: Same as first input
  Sum8 : Sum  Inputs=+-  InputSameDT=on  SaturateOnIntegerOverflow=on  OutDataTypeStr=Inherit: Same as first input
  Sum9 : Sum  Inputs=|+-  InputSameDT=on  SaturateOnIntegerOverflow=on  OutDataTypeStr=Inherit: Same as first input
  negative half : Saturate  UpperLimit=0  LowerLimit=-inf  ZeroCross=off
  positive half : Saturate  UpperLimit=inf  LowerLimit=0  ZeroCross=off
  LStimSOL : Outport  OutputWhenDisabled=reset  InitialOutput=0
  LStimTA : Outport  Port=2  OutputWhenDisabled=reset  InitialOutput=0
  LStimGAS : Outport  Port=3  OutputWhenDisabled=reset  InitialOutput=0
  LStimVAS : Outport  Port=4  OutputWhenDisabled=reset  InitialOutput=0
  LStimHAM : Outport  Port=5  OutputWhenDisabled=reset  InitialOutput=0
  LStimGLU : Outport  Port=6  OutputWhenDisabled=reset  InitialOutput=0
  LStimHFL : Outport  Port=7  OutputWhenDisabled=reset  InitialOutput=0
  Delta_Theta : Outport  Port=8  InitialOutput=0
  wires:
  Sum1/1 -> Sum2/1
  FB Gain/1 -> Sum2/2
  FB Gain1/1 -> Product1/2
  Saturation4/1 -> FB Gain1/1
  dTheta [rad/s]/1 -> FB Gain10/1
  Stimulation Bias6/1 -> Sum9/2
  Theta/1 -> Sum9/1
  negative half/1 -> Sum11/1
  Sum9/1 -> FB Gain11/1, Delta_Theta/1
  LFmSOL/1 -> FB Gain4/1, FB Gain3/1
  LFmVAS/1 -> FB Gain/1
  RdxThigh [N]/1 -> Saturation4/1
  LFmGAS/1 -> FB Gain2/1
  FB Gain4/1 -> Sum6/2
  Sum6/1 -> LStimSOL/1
  Stimulation Bias1/1 -> Sum3/1
  Sum3/1 -> LStimGAS/1
  FB Gain2/1 -> Sum3/2
  positive half/1 -> Sum10/2
  Stimulation Bias7/1 -> Sum10/1, Sum11/2
  FB Gain11/1 -> Sum12/1
  FB Gain10/1 -> Sum12/2
  Sum12/1 -> positive half/1, negative half/1
  Sum13/1 -> LStimHFL/1
  Product1/1 -> Sum1/1
  Saturation1/1 -> Sum13/1
  Saturation2/1 -> FB Gain6/1
  Sum11/1 -> Divide1/2
  Sum10/1 -> Divide/1
  LdxThigh [N]/1 -> Saturation2/1
  Divide1/1 -> Saturation1/1
  Gain1/1 -> LStimGLU/1
  FB Gain3/1 -> Sum4/2
  Stimulation Bias2/1 -> Sum4/1
  Sum4/1 -> Sum7/1
  Sum7/1 -> LStimTA/1
  FB Gain8/1 -> Sum7/2
  LLceTA/1 -> FB Gain8/1
  Stimulation Bias/1 -> Sum1/2
  Sum2/1 -> Sum14/1
  Sum14/1 -> LStimVAS/1
  Gain3/1 -> Sum13/2
  Stimulation Bias3/1 -> Sum6/1
  FB Gain6/1 -> Divide/2, Divide1/1
  Divide/1 -> Saturation3/1
  Sum8/1 -> Gain1/1
  Gain4/1 -> Sum8/2
  Saturation3/1 -> Sum8/1, Gain/1
  Gain2/1 -> Sum14/2
  LKneeState/1 -> Gain2/1
  RonL/1 -> Product1/1, Gain3/1, Gain4/1
  Gain/1 -> LStimHAM/1

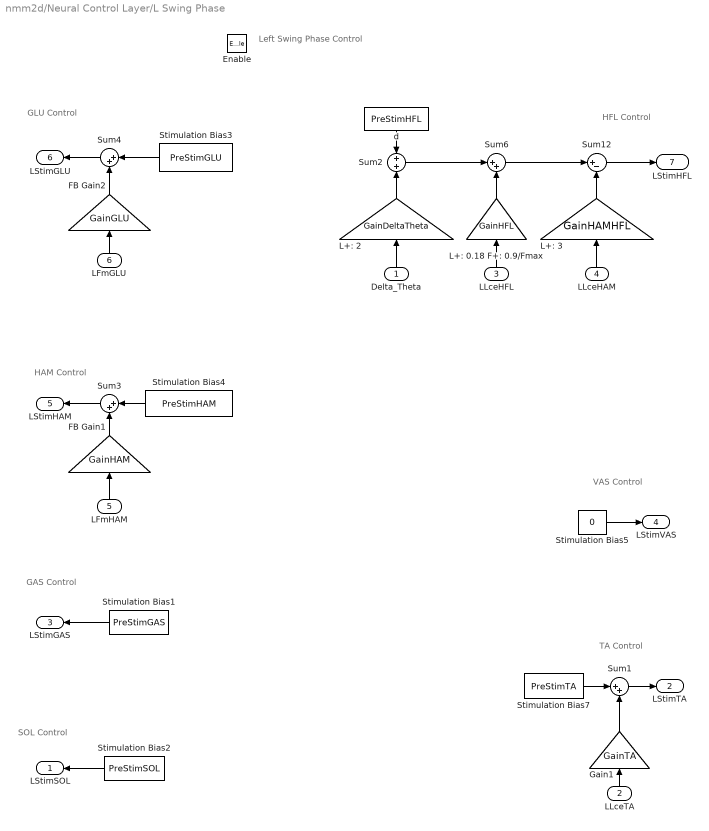
== system nmm2d/Neural Control Layer/L Swing Phase ==
  note: SOL Control
  note: GAS Control
  note: VAS Control
  note: Left Swing Phase Control
  note: HAM Control
  note: GLU Control
  note: HFL Control
  note: TA Control
  Delta_Theta : Inport
  LLceTA : Inport  Port=2
  LLceHFL : Inport  Port=3
  LLceHAM : Inport  Port=4
  LFmHAM : Inport  Port=5
  LFmGLU : Inport  Port=6
  Enable : EnablePort  StatesWhenEnabling=reset
  FB Gain1 : Gain  Gain=GainHAM  SaturateOnIntegerOverflow=on  OutDataTypeStr=Inherit: Same as input  ParamDataTypeStr=Inherit: Same as input
  FB Gain2 : Gain  Gain=GainGLU  SaturateOnIntegerOverflow=on  OutDataTypeStr=Inherit: Same as input  ParamDataTypeStr=Inherit: Same as input
  Gain1 : Gain  Gain=GainTA
  L+: 0.18 F+: 0.9/Fmax : Gain  Gain=GainHFL  SaturateOnIntegerOverflow=on  OutDataTypeStr=Inherit: Same as input  ParamDataTypeStr=Inherit: Same as input
  L+: 2 : Gain  Gain=GainDeltaTheta  SaturateOnIntegerOverflow=on  OutDataTypeStr=Inherit: Same as input  ParamDataTypeStr=Inherit: Same as input
  L+: 3 : Gain  Gain=GainHAMHFL  SaturateOnIntegerOverflow=on  OutDataTypeStr=Inherit: Same as input  ParamDataTypeStr=Inherit: Same as input
  Stimulation Bias1 : Constant  Value=PreStimGAS
  Stimulation Bias2 : Constant  Value=PreStimSOL
  Stimulation Bias3 : Constant  Value=PreStimGLU
  Stimulation Bias4 : Constant  Value=PreStimHAM
  Stimulation Bias5 : Constant  Value=0
  Stimulation Bias7 : Constant  Value=PreStimTA
  Sum{1,3..4,6} (4 alike) : Sum  Inputs=|++  InputSameDT=on  SaturateOnIntegerOverflow=on  OutDataTypeStr=Inherit: Same as first input
  Sum12 : Sum  Inputs=|+-  InputSameDT=on  SaturateOnIntegerOverflow=on  OutDataTypeStr=Inherit: Same as first input
  Sum2 : Sum  InputSameDT=on  SaturateOnIntegerOverflow=on  OutDataTypeStr=Inherit: Same as first input
  d : Constant  Value=PreStimHFL
  LStimSOL : Outport  OutputWhenDisabled=reset  InitialOutput=0
  LStimTA : Outport  Port=2  OutputWhenDisabled=reset  InitialOutput=0
  LStimGAS : Outport  Port=3  OutputWhenDisabled=reset  InitialOutput=0
  LStimVAS : Outport  Port=4  OutputWhenDisabled=reset  InitialOutput=0
  LStimHAM : Outport  Port=5  OutputWhenDisabled=reset  InitialOutput=0
  LStimGLU : Outport  Port=6  OutputWhenDisabled=reset  InitialOutput=0
  LStimHFL : Outport  Port=7  OutputWhenDisabled=reset  InitialOutput=0
  wires:
  Stimulation Bias1/1 -> LStimGAS/1
  Stimulation Bias2/1 -> LStimSOL/1
  FB Gain1/1 -> Sum3/2
  Stimulation Bias4/1 -> Sum3/1
  LLceTA/1 -> Gain1/1
  Stimulation Bias7/1 -> Sum1/1
  Sum1/1 -> LStimTA/1
  Gain1/1 -> Sum1/2
  Sum3/1 -> LStimHAM/1
  Stimulation Bias5/1 -> LStimVAS/1
  LLceHFL/1 -> L+: 0.18 F+: 0.9/Fmax/1
  L+: 0.18 F+: 0.9/Fmax/1 -> Sum6/2
  LLceHAM/1 -> L+: 3/1
  L+: 3/1 -> Sum12/2
  Sum6/1 -> Sum12/1
  Delta_Theta/1 -> L+: 2/1
  d/1 -> Sum2/1
  Sum2/1 -> Sum6/1
  L+: 2/1 -> Sum2/2
  FB Gain2/1 -> Sum4/2
  LFmGLU/1 -> FB Gain2/1
  Stimulation Bias3/1 -> Sum4/1
  Sum4/1 -> LStimGLU/1
  LFmHAM/1 -> FB Gain1/1
  Sum12/1 -> LStimHFL/1

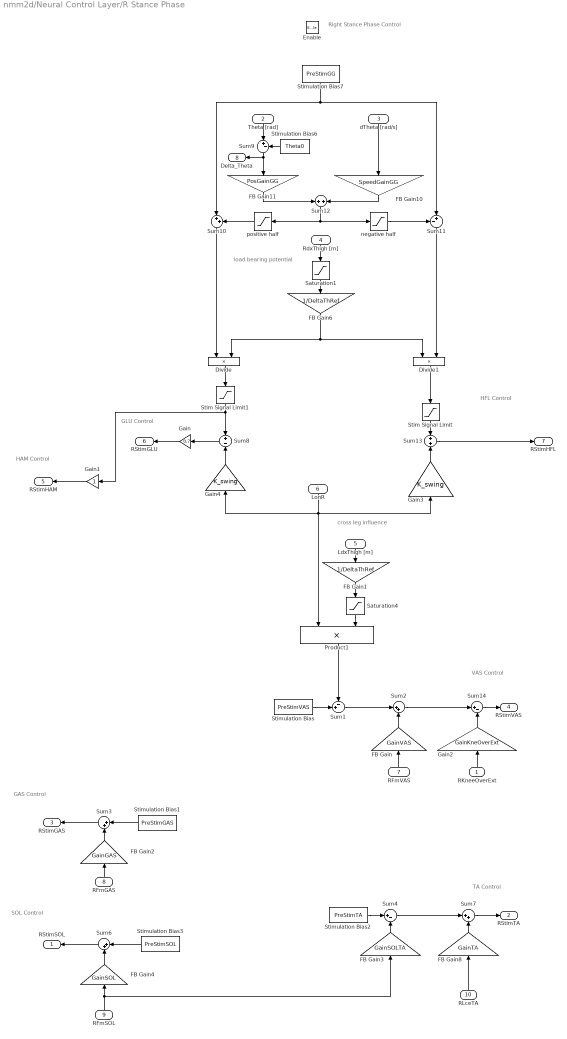
== system nmm2d/Neural Control Layer/R Stance Phase ==
  note: HFL Control
  note: GLU Control
  note: SOL Control
  note: TA Control
  note: GAS Control
  note: VAS Control
  note: Right Stance Phase Control
  note: HAM Control
  note: cross leg influence
  note: load bearing potential
  RKneeOverExt : Inport
  Theta [rad] : Inport  Port=2
  dTheta [rad/s] : Inport  Port=3
  RdxThigh [m] : Inport  Port=4
  LdxThigh [m] : Inport  Port=5
  LonR : Inport  Port=6
  RFmVAS : Inport  Port=7
  RFmGAS : Inport  Port=8
  RFmSOL : Inport  Port=9
  RLceTA : Inport  Port=10
  Enable : EnablePort  StatesWhenEnabling=reset
  Divide : Product
  Divide1 : Product
  FB Gain : Gain  Gain=GainVAS  SaturateOnIntegerOverflow=on  OutDataTypeStr=Inherit: Same as input  ParamDataTypeStr=Inherit: Same as input
  FB Gain1 : Gain  Gain=1/DeltaThRef  SaturateOnIntegerOverflow=on  OutDataTypeStr=Inherit: Same as input  ParamDataTypeStr=Inherit: Same as input
  FB Gain10 : Gain  Gain=SpeedGainGG  SaturateOnIntegerOverflow=on  OutDataTypeStr=Inherit: Same as input  ParamDataTypeStr=Inherit: Same as input
  FB Gain11 : Gain  Gain=PosGainGG  SaturateOnIntegerOverflow=on  OutDataTypeStr=Inherit: Same as input  ParamDataTypeStr=Inherit: Same as input
  FB Gain2 : Gain  Gain=GainGAS  SaturateOnIntegerOverflow=on  OutDataTypeStr=Inherit: Same as input  ParamDataTypeStr=Inherit: Same as input
  FB Gain3 : Gain  Gain=GainSOLTA  SaturateOnIntegerOverflow=on  OutDataTypeStr=Inherit: Same as input  ParamDataTypeStr=Inherit: Same as input
  FB Gain4 : Gain  Gain=GainSOL  SaturateOnIntegerOverflow=on  OutDataTypeStr=Inherit: Same as input  ParamDataTypeStr=Inherit: Same as input
  FB Gain6 : Gain  Gain=1/DeltaThRef  SaturateOnIntegerOverflow=on  OutDataTypeStr=Inherit: Same as input  ParamDataTypeStr=Inherit: Same as input
  FB Gain8 : Gain  Gain=GainTA  SaturateOnIntegerOverflow=on  OutDataTypeStr=Inherit: Same as input  ParamDataTypeStr=Inherit: Same as input
  Gain : Gain  Gain=0.7
  Gain1 : Gain
  Gain2 : Gain  Gain=GainKneOverExt
  Gain3 : Gain  Gain=K_swing
  Gain4 : Gain  Gain=K_swing
  Product1 : Product  RndMeth=Zero
  Saturation1 : Saturate  UpperLimit=inf  LowerLimit=0  ZeroCross=off
  Saturation4 : Saturate  UpperLimit=inf  LowerLimit=0  ZeroCross=off
  Stim Signal Limit : Saturate  UpperLimit=1  LowerLimit=0  ZeroCross=off
  Stim Signal Limit1 : Saturate  UpperLimit=1  LowerLimit=0  ZeroCross=off
  Stimulation Bias : Constant  Value=PreStimVAS
  Stimulation Bias1 : Constant  Value=PreStimGAS
  Stimulation Bias2 : Constant  Value=PreStimTA
  Stimulation Bias3 : Constant  Value=PreStimSOL
  Stimulation Bias6 : Constant  Value=Theta0
  Stimulation Bias7 : Constant  Value=PreStimGG
  Sum1 : Sum  Inputs=-+|  InputSameDT=on  SaturateOnIntegerOverflow=on  OutDataTypeStr=Inherit: Same as first input
  Sum{2..3,6..7,10} (5 alike) : Sum  Inputs=|++  InputSameDT=on  SaturateOnIntegerOverflow=on  OutDataTypeStr=Inherit: Same as first input
  Sum11 : Sum  Inputs=-+|  InputSameDT=on  SaturateOnIntegerOverflow=on  OutDataTypeStr=Inherit: Same as first input
  Sum12 : Sum  InputSameDT=on  SaturateOnIntegerOverflow=on  OutDataTypeStr=Inherit: Same as first input
  Sum13 : Sum  InputSameDT=on  SaturateOnIntegerOverflow=on  OutDataTypeStr=Inherit: Same as first input
  Sum14 : Sum  Inputs=|+-  InputSameDT=on  SaturateOnIntegerOverflow=on  OutDataTypeStr=Inherit: Same as first input
  Sum4 : Sum  Inputs=|+-  InputSameDT=on  SaturateOnIntegerOverflow=on  OutDataTypeStr=Inherit: Same as first input
  Sum8 : Sum  Inputs=+-  InputSameDT=on  SaturateOnIntegerOverflow=on  OutDataTypeStr=Inherit: Same as first input
  Sum9 : Sum  Inputs=|+-  InputSameDT=on  SaturateOnIntegerOverflow=on  OutDataTypeStr=Inherit: Same as first input
  negative half : Saturate  UpperLimit=0  LowerLimit=-inf  ZeroCross=off
  positive half : Saturate  UpperLimit=inf  LowerLimit=0  ZeroCross=off
  RStimSOL : Outport  OutputWhenDisabled=reset  InitialOutput=0
  RStimTA : Outport  Port=2  OutputWhenDisabled=reset  InitialOutput=0
  RStimGAS : Outport  Port=3  OutputWhenDisabled=reset  InitialOutput=0
  RStimVAS : Outport  Port=4  OutputWhenDisabled=reset  InitialOutput=0
  RStimHAM : Outport  Port=5  OutputWhenDisabled=reset  InitialOutput=0
  RStimGLU : Outport  Port=6  OutputWhenDisabled=reset  InitialOutput=0
  RStimHFL : Outport  Port=7  OutputWhenDisabled=reset  InitialOutput=0
  Delta_Theta : Outport  Port=8  InitialOutput=0
  wires:
  Saturation4/1 -> Product1/2
  dTheta [rad/s]/1 -> FB Gain10/1
  Stimulation Bias6/1 -> Sum9/2
  Theta [rad]/1 -> Sum9/1
  negative half/1 -> Sum11/1
  Sum9/1 -> FB Gain11/1, Delta_Theta/1
  RFmSOL/1 -> FB Gain4/1, FB Gain3/1
  RFmVAS/1 -> FB Gain/1
  LdxThigh [m]/1 -> FB Gain1/1
  RFmGAS/1 -> FB Gain2/1
  FB Gain4/1 -> Sum6/2
  Sum6/1 -> RStimSOL/1
  FB Gain3/1 -> Sum4/2
  Stimulation Bias2/1 -> Sum4/1
  Sum3/1 -> RStimGAS/1
  FB Gain2/1 -> Sum3/2
  positive half/1 -> Sum10/2
  Stimulation Bias7/1 -> Sum10/1, Sum11/2
  FB Gain11/1 -> Sum12/1
  FB Gain10/1 -> Sum12/2
  Sum12/1 -> positive half/1, negative half/1
  Sum13/1 -> RStimHFL/1
  Product1/1 -> Sum1/1
  Stim Signal Limit/1 -> Sum13/1
  RdxThigh [m]/1 -> Saturation1/1
  Sum10/1 -> Divide/1
  Sum11/1 -> Divide1/2
  Saturation1/1 -> FB Gain6/1
  Divide1/1 -> Stim Signal Limit/1
  FB Gain/1 -> Sum2/2
  Sum4/1 -> Sum7/1
  Sum7/1 -> RStimTA/1
  RLceTA/1 -> FB Gain8/1
  FB Gain8/1 -> Sum7/2
  RKneeOverExt/1 -> Gain2/1
  Sum14/1 -> RStimVAS/1
  Gain/1 -> RStimGLU/1
  Stimulation Bias3/1 -> Sum6/1
  Stimulation Bias1/1 -> Sum3/1
  Gain3/1 -> Sum13/2
  FB Gain6/1 -> Divide/2, Divide1/1
  Divide/1 -> Stim Signal Limit1/1
  Stim Signal Limit1/1 -> Sum8/1, Gain1/1
  Stimulation Bias/1 -> Sum1/2
  Sum1/1 -> Sum2/1
  Sum2/1 -> Sum14/1
  Gain2/1 -> Sum14/2
  Gain4/1 -> Sum8/2
  Sum8/1 -> Gain/1
  LonR/1 -> Product1/1, Gain3/1, Gain4/1
  FB Gain1/1 -> Saturation4/1
  Gain1/1 -> RStimHAM/1

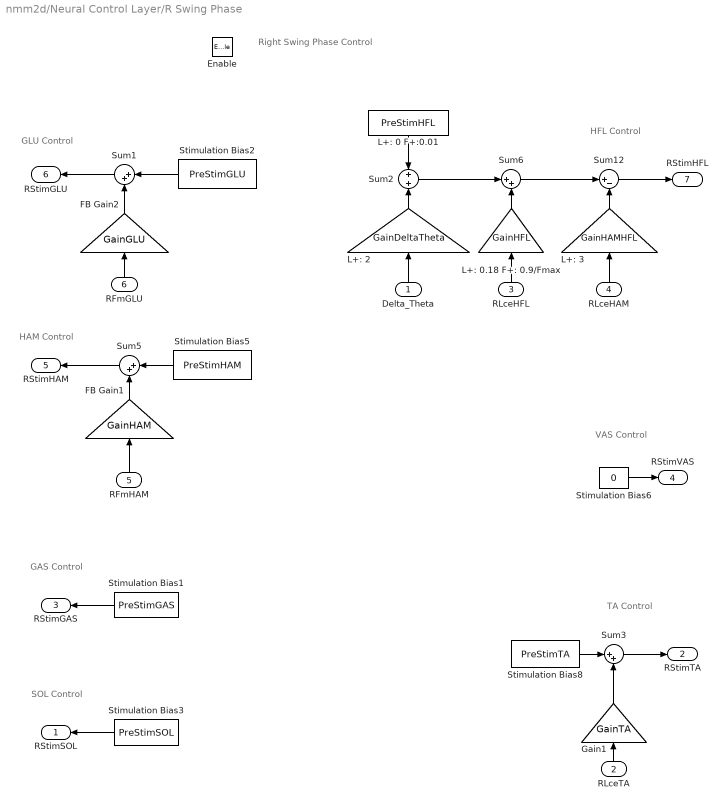
== system nmm2d/Neural Control Layer/R Swing Phase ==
  note: Right Swing Phase Control
  note: VAS Control
  note: GAS Control
  note: TA Control
  note: SOL Control
  note: GLU Control
  note: HFL Control
  note: HAM Control
  Delta_Theta : Inport
  RLceTA : Inport  Port=2
  RLceHFL : Inport  Port=3
  RLceHAM : Inport  Port=4
  RFmHAM : Inport  Port=5
  RFmGLU : Inport  Port=6
  Enable : EnablePort  StatesWhenEnabling=reset
  FB Gain1 : Gain  Gain=GainHAM  SaturateOnIntegerOverflow=on  OutDataTypeStr=Inherit: Same as input  ParamDataTypeStr=Inherit: Same as input
  FB Gain2 : Gain  Gain=GainGLU  SaturateOnIntegerOverflow=on  OutDataTypeStr=Inherit: Same as input  ParamDataTypeStr=Inherit: Same as input
  Gain1 : Gain  Gain=GainTA
  L+: 0 F+:0.01 : Constant  Value=PreStimHFL
  L+: 0.18 F+: 0.9/Fmax : Gain  Gain=GainHFL  SaturateOnIntegerOverflow=on  OutDataTypeStr=Inherit: Same as input  ParamDataTypeStr=Inherit: Same as input
  L+: 2 : Gain  Gain=GainDeltaTheta  SaturateOnIntegerOverflow=on  OutDataTypeStr=Inherit: Same as input  ParamDataTypeStr=Inherit: Same as input
  L+: 3 : Gain  Gain=GainHAMHFL  SaturateOnIntegerOverflow=on  OutDataTypeStr=Inherit: Same as input  ParamDataTypeStr=Inherit: Same as input
  Stimulation Bias1 : Constant  Value=PreStimGAS
  Stimulation Bias2 : Constant  Value=PreStimGLU
  Stimulation Bias3 : Constant  Value=PreStimSOL
  Stimulation Bias5 : Constant  Value=PreStimHAM
  Stimulation Bias6 : Constant  Value=0
  Stimulation Bias8 : Constant  Value=PreStimTA
  Sum{1,3,5..6} (4 alike) : Sum  Inputs=|++  InputSameDT=on  SaturateOnIntegerOverflow=on  OutDataTypeStr=Inherit: Same as first input
  Sum12 : Sum  Inputs=|+-  InputSameDT=on  SaturateOnIntegerOverflow=on  OutDataTypeStr=Inherit: Same as first input
  Sum2 : Sum  InputSameDT=on  SaturateOnIntegerOverflow=on  OutDataTypeStr=Inherit: Same as first input
  RStimSOL : Outport  OutputWhenDisabled=reset  InitialOutput=0
  RStimTA : Outport  Port=2  OutputWhenDisabled=reset  InitialOutput=0
  RStimGAS : Outport  Port=3  OutputWhenDisabled=reset  InitialOutput=0
  RStimVAS : Outport  Port=4  OutputWhenDisabled=reset  InitialOutput=0
  RStimHAM : Outport  Port=5  OutputWhenDisabled=reset  InitialOutput=0
  RStimGLU : Outport  Port=6  OutputWhenDisabled=reset  InitialOutput=0
  RStimHFL : Outport  Port=7  OutputWhenDisabled=reset  InitialOutput=0
  wires:
  Stimulation Bias1/1 -> RStimGAS/1
  Stimulation Bias3/1 -> RStimSOL/1
  FB Gain1/1 -> Sum5/2
  Stimulation Bias5/1 -> Sum5/1
  RLceTA/1 -> Gain1/1
  Stimulation Bias8/1 -> Sum3/1
  Sum3/1 -> RStimTA/1
  Gain1/1 -> Sum3/2
  Sum5/1 -> RStimHAM/1
  Stimulation Bias6/1 -> RStimVAS/1
  L+: 0.18 F+: 0.9/Fmax/1 -> Sum6/2
  RLceHAM/1 -> L+: 3/1
  Sum6/1 -> Sum12/1
  RLceHFL/1 -> L+: 0.18 F+: 0.9/Fmax/1
  L+: 0 F+:0.01/1 -> Sum2/1
  Sum2/1 -> Sum6/1
  L+: 2/1 -> Sum2/2
  Delta_Theta/1 -> L+: 2/1
  L+: 3/1 -> Sum12/2
  FB Gain2/1 -> Sum1/2
  RFmGLU/1 -> FB Gain2/1
  Stimulation Bias2/1 -> Sum1/1
  Sum1/1 -> RStimGLU/1
  RFmHAM/1 -> FB Gain1/1
  Sum12/1 -> RStimHFL/1

== system nmm2d/Body Mechanics Layer/Left Ball Contact/Ground Friction Model ==
  note: Horizontal Ground Friction Model
  note: Vertical Ground Stiction Model
  dy [m] : Inport
  vy [m/s] : Inport  Port=2
  x [m] : Inport  Port=3
  vx [m/s] : Inport  Port=4
  vBelt [m/s] : Inport  Port=5
  Contact! : EnablePort  StatesWhenEnabling=reset
  Data Type Conversion : DataTypeConversion  OutDataTypeStr=double  SaturateOnIntegerOverflow=off  RndMeth=Floor
  Friction Switch : Subsystem
  Gain3 : Gain  Gain=k_gy
  Gain4 : Gain  Gain=1/v_gy_max
  Logical Operator : Logic  Operator=NOT  AllPortsSameDT=off  OutDataTypeStr=boolean
  Mux1 : Mux  Inputs=2
  Sum1 : Sum
  X-Axis Kinetic Friction Model : Subsystem
  X-Axis Static Friction Model : Subsystem
  Y-Axis Ground Force : Fcn  Expr="- u(1)  *  (1-u(2)) * (u(2)<1)"
  Fy_Ground[N] : Outport  OutputWhenDisabled=reset  InitialOutput=0
      settings: AttributesFormatString=initial = '%<InitialOutput>'\nwhen disabled = '%<OutputWhenDisabled>'
  Fx_Friction [N] : Outport  Port=2  OutputWhenDisabled=reset  InitialOutput=0
      settings: AttributesFormatString=initial = '%<InitialOutput>'\nwhen\ndisabled\n'%<OutputWhenDisabled>'
  Stiction! : Outport  Port=3  OutputWhenDisabled=reset  InitialOutput=0
      settings: AttributesFormatString=initial = '%<InitialOutput>'\nwhen\ndisabled\n'%<OutputWhenDisabled>'
  wires:
  Y-Axis Ground Force/1 -> X-Axis Kinetic Friction Model/4(F_Normal [N]), X-Axis Static Friction Model/1(F_Normal [N]), Fy_Ground[N]/1
  dy [m]/1 -> Gain3/1
  vy [m/s]/1 -> Gain4/1
  x [m]/1 -> X-Axis Kinetic Friction Model/1(pos [m]), X-Axis Static Friction Model/3(pos [m])
  vx [m/s]/1 -> X-Axis Static Friction Model/4(vel [m/s]), X-Axis Kinetic Friction Model/2(vel [m/s])
  X-Axis Kinetic Friction Model/1(initial posFP [m]) -> X-Axis Static Friction Model/5(initial posFP [m])
  X-Axis Kinetic Friction Model/3(F_Slide [N]) -> Sum1/2
  X-Axis Static Friction Model/1(F_Stick [N]) -> Sum1/1
  Sum1/1 -> Fx_Friction [N]/1
  Friction Switch/1(Stiction) -> X-Axis Static Friction Model/Enable, Logical Operator/1, Data Type Conversion/1
  X-Axis Static Friction Model/2(Sliding!) -> Friction Switch/1(Slide!)
  X-Axis Kinetic Friction Model/2(Stiction!) -> Friction Switch/2(Stick!)
  Logical Operator/1 -> X-Axis Kinetic Friction Model/Enable
  Data Type Conversion/1 -> Stiction!/1
  Mux1/1 -> Y-Axis Ground Force/1
  Gain3/1 -> Mux1/1
  Gain4/1 -> Mux1/2
  vBelt [m/s]/1 -> X-Axis Kinetic Friction Model/3(vBelt [m/s]), X-Axis Static Friction Model/2(vBelt [m/s])

== system nmm2d/Body Mechanics Layer/Left Heel Contact/Ground Friction Model ==
  note: Vertical Ground Stiction Model
  note: Horizontal Ground Friction Model
  dy [m] : Inport
  vy [m/s] : Inport  Port=2
  x [m] : Inport  Port=3
  vx [m/s] : Inport  Port=4
  vBelt [m/s] : Inport  Port=5
  Contact! : EnablePort  StatesWhenEnabling=reset
  Data Type Conversion : DataTypeConversion  OutDataTypeStr=double  SaturateOnIntegerOverflow=off  RndMeth=Floor
  Friction Switch : Subsystem
  Gain3 : Gain  Gain=k_gy
  Gain4 : Gain  Gain=1/v_gy_max
  Logical Operator : Logic  Operator=NOT  AllPortsSameDT=off  OutDataTypeStr=boolean
  Mux1 : Mux  Inputs=2
  Sum1 : Sum
  X-Axis Kinetic Friction Model : Subsystem
  X-Axis Static Friction Model : Subsystem
  Y-Axis Ground Force : Fcn  Expr="- u(1)  *  (1-u(2)) * (u(2)<1)"
  Fy_Ground[N] : Outport  OutputWhenDisabled=reset  InitialOutput=0
      settings: AttributesFormatString=initial = '%<InitialOutput>'\nwhen disabled = '%<OutputWhenDisabled>'
  Fx_Friction [N] : Outport  Port=2  OutputWhenDisabled=reset  InitialOutput=0
      settings: AttributesFormatString=initial = '%<InitialOutput>'\nwhen\ndisabled\n'%<OutputWhenDisabled>'
  Stiction! : Outport  Port=3  OutputWhenDisabled=reset  InitialOutput=0
      settings: AttributesFormatString=initial = '%<InitialOutput>'\nwhen\ndisabled\n'%<OutputWhenDisabled>'
  wires:
  vBelt [m/s]/1 -> X-Axis Static Friction Model/2(vBelt [m/s]), X-Axis Kinetic Friction Model/3(vBelt [m/s])
  Gain4/1 -> Mux1/2
  Gain3/1 -> Mux1/1
  Mux1/1 -> Y-Axis Ground Force/1
  Data Type Conversion/1 -> Stiction!/1
  Logical Operator/1 -> X-Axis Kinetic Friction Model/Enable
  X-Axis Kinetic Friction Model/2(Stiction!) -> Friction Switch/2(Stick!)
  X-Axis Static Friction Model/2(Sliding!) -> Friction Switch/1(Slide!)
  Friction Switch/1(Stiction) -> Data Type Conversion/1, Logical Operator/1, X-Axis Static Friction Model/Enable
  Sum1/1 -> Fx_Friction [N]/1
  X-Axis Static Friction Model/1(F_Stick [N]) -> Sum1/1
  X-Axis Kinetic Friction Model/3(F_Slide [N]) -> Sum1/2
  X-Axis Kinetic Friction Model/1(initial posFP [m]) -> X-Axis Static Friction Model/5(initial posFP [m])
  vx [m/s]/1 -> X-Axis Kinetic Friction Model/2(vel [m/s]), X-Axis Static Friction Model/4(vel [m/s])
  x [m]/1 -> X-Axis Static Friction Model/3(pos [m]), X-Axis Kinetic Friction Model/1(pos [m])
  vy [m/s]/1 -> Gain4/1
  dy [m]/1 -> Gain3/1
  Y-Axis Ground Force/1 -> Fy_Ground[N]/1, X-Axis Static Friction Model/1(F_Normal [N]), X-Axis Kinetic Friction Model/4(F_Normal [N])
